simulink model "WindFarmDFIG"  (R2024a)
settings: Solver=FixedStepDiscrete  StartTime=0.0  StopTime=0.2  RelTol=1e-3
PreLoadFcn:
  | Ts=5e-6;
InitFcn:
  | xInitial = WindFarmDFIGInit;
  | Ts=5e-6;
undefined symbols (not defined in the file): D1, D11, Delta, DiscIntNeverNeededParam, find_system, level
libraries: powerlib_extras x38, spsThreePhaseVIMeasurementLib x6, simulink_extras x6, spsThreePhaseTransformerTwoWindingsLib x3, spsSeriesRLCBranchLib x2, spsUniversalBridgeLib x2, spsGroundLib x2, spsThreePhaseProgrammableVoltageSourceLib x1, spsThreePhaseMutualInductanceZ1Z0Lib x1, spsThreePhasePISectionLineLib x1, spsAsynchronousMachinepuUnitsLib x1, spsThreePhaseSeriesRLCBranchLib x1
(part 2 of 3)

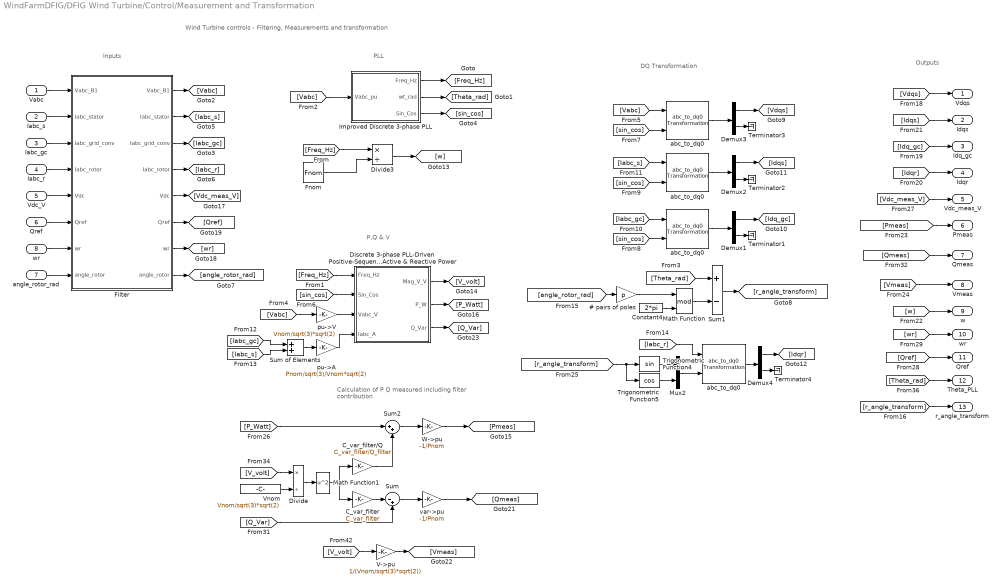
== system WindFarmDFIG/DFIG Wind Turbine/Control/Measurement and Transformation ==
  note: DQ Transformation
  note: P,Q & V
  note: PLL
  note: Inputs
  note: Outputs
  note: Calculation of P Q measured
      | including filter contribution
  note: Wind Turbine controls - Filtering, Measurements and transformation
  Vabc : Inport
  Iabc_s : Inport  Port=2
  Iabc_gc : Inport  Port=3
  Iabc_r : Inport  Port=4
  Vdc_V : Inport  Port=5
  Qref : Inport  Port=6
  angle_rotor_rad : Inport  Port=7
  wr : Inport  Port=8
  "   abc_to_dq0    " : powerlib_extras/Measurements/abc_to_dq0 Transformation
  " Improved Discrete 3-phase PLL" : Subsystem  mask(Discrete 3-phase PLL){Fmin=0.75*Fnom, Par_Init=[0 Fnom], ParK=[5 3.2 1 50], Ts=Ts}
      mask prompts: Fmin "Minimum frequency (Hz):"; Par_Init "Initial inputs:[ Phase(degrees)   Frequency(Hz) ]"; ParK "Regulator gains [ Kp1 Kp2  Ki1  Ki2 ]"; Ts "Sample time:"
      mask help:
      | This Phase Locked Loop (PLL) system can be used  to synchronize on a set of variable frequency, three-phase sinusoidal signals.
      |
      | Input 1: Vector containing the normalized
      |              three-phase signals [Va Vb Vc]
      | Output 1:  Measured frequency (Hz) = w/(2pi)
      | Output 2:  Ramp w.t   varying between  0 and 2*pi,
      | synchronized on zero crossings of the fundamental (positive-sequence) of phase A.
      | Output 3: Vector [sin(wt) cos(wt)]
      mask init:
      | Kp1=ParK(1);
      | Kp2=ParK(2);
      | Ki1=ParK(3);
      | Ki2=ParK(4);
      | Phase_Init=Par_Init(1);
      | Finit=Par_Init(2);
      | power_initmask();
      settings: OpenFcn=power_openblockproxy();
  # pairs of poles : Gain  Gain=p  SaturateOnIntegerOverflow=on  OutDataTypeStr=Inherit: Same as input  ParamDataTypeStr=Inherit: Same as input
  C_var_filter : Gain  Gain=C_var_filter  SaturateOnIntegerOverflow=on  OutDataTypeStr=Inherit: Same as input  ParamDataTypeStr=Inherit: Same as input
  C_var_filter/Q : Gain  Gain=C_var_filter/Q_filter  SaturateOnIntegerOverflow=on  OutDataTypeStr=Inherit: Same as input  ParamDataTypeStr=Inherit: Same as input
  Constant4 : Constant  Value=2*pi
  Demux{1..4} (4 alike) : Demux  Outputs=[2 1]
      settings: DisplayOption=none
  Discrete 3-phase PLL-Driven Positive-Sequence Active & Reactive Power : Subsystem  mask(Discrete 3-phase PLL-Driven Positive-Sequence Active & Reactive Power){Finit=Fnom, Fmin=Fnom*45/60, Par_Vinit=[Vnom/sqrt(3)*sqrt(2) 30], Par_Iinit=[Pnom/sqrt(3)/Vnom*sqrt(2) -10], Ts=Ts}
      mask prompts: Finit "Initial frequency (Hz):"; Fmin "Minimum frequency (Hz):"; Par_Vinit "Voltage initial input: [ Mag  Phase(Degrees) ]"; Par_Iinit "Current initial input: [ Mag  Phase(Degrees) ]"; Ts "Sample time:"
      mask help:
      | This discrete block measures the 3-phase active power P and reactive power Q  associated with a periodic set of 3-phase voltages and currents which may contain harmonics. P and Q are calculated by evaluating the fundamental values (positive-sequence) of the input voltages and currents with a running window over one cycle of the specified frequency (port Freq).
      |  Input port "Sin_Cos" (a two-dimension signal) provides the reference frame required for the computation.
      |
      | input 1: must give the frequency of the fundamental (Hz)
      | Input 2: must contain a  [sin(wt)  cos(wt)] two dimension signal , where w is the rotation speed (rad/s) of the reference frame used for the computation..
      | input 3: Vectorized 3-phase  instantaneous voltage (Vabc)
      | input 4: Vectorized 3-phase instantaneous current (Iabc)
      |
      | Output 1: Vector [Mag_V Mag_I] of the fundamental values (Magnitude) of the voltage & current (peak values of the positive-sequence)
      | Output 2: 3-phase PQ measurement vector [P(W) Q (var)] evaluated at the specified frequency. Current flowing into an RL circuit will produce  positive active and reactive powers.
      |
      | For the first cycle of simulation, the outputs are held constant using the values specified by the parameters "Initial input".
      | he value of the parameter "Minimum frequency" is used to determine the buffer size of the "Variable Transport Delay" block found inside this subsystem.
      mask init:
      | power_initmask();
      settings: OpenFcn=power_openblockproxy();
  Divide : Product  Inputs=*/
  Divide3 : Product  Inputs=*/
  Filter : Subsystem  mask{Freq=Freq_filter, Zeta1=Zeta_filter, Ts=Ts}
      mask prompts: Freq "Cut-off frequency (Hz):"; Zeta1 "Damping factor Zeta:"; Ts "Sample time"
  Fnom : Constant  Value=Fnom
  Math Function : Math  Operator=mod  SignedPower=on
  Math Function1 : Math  Operator=square  SignedPower=on
  Mux2 : Mux  Inputs=2
  Sum : Sum  Inputs=|-+
  Sum of Elements : Sum
  Sum1 : Sum  Inputs=+-  InputSameDT=on  SaturateOnIntegerOverflow=on  OutDataTypeStr=Inherit: Same as first input
  Sum2 : Sum  Inputs=|++
  Terminator{1..4} (4 alike) : Terminator
  Trigonometric Function4 : Trigonometry
  Trigonometric Function5 : Trigonometry  Operator=cos
  V->pu : Gain  Gain=1/(Vnom/sqrt(3)*sqrt(2))  SaturateOnIntegerOverflow=on  OutDataTypeStr=Inherit: Same as input  ParamDataTypeStr=Inherit: Same as input
  Vnom : Constant  Value=Vnom/sqrt(3)*sqrt(2)
  W->pu : Gain  Gain=-1/Pnom  SaturateOnIntegerOverflow=on  OutDataTypeStr=Inherit: Same as input  ParamDataTypeStr=Inherit: Same as input
  abc_to_dq0 : powerlib_extras/Measurements/abc_to_dq0 Transformation
  "abc_to_dq0 " : powerlib_extras/Measurements/abc_to_dq0 Transformation
  "abc_to_dq0  " : powerlib_extras/Measurements/abc_to_dq0 Transformation
  pu->A : Gain  Gain=Pnom/sqrt(3)/Vnom*sqrt(2)  SaturateOnIntegerOverflow=on  OutDataTypeStr=Inherit: Same as input  ParamDataTypeStr=Inherit: Same as input
  pu->V : Gain  Gain=Vnom/sqrt(3)*sqrt(2)  SaturateOnIntegerOverflow=on  OutDataTypeStr=Inherit: Same as input  ParamDataTypeStr=Inherit: Same as input
  "var->pu " : Gain  Gain=-1/Pnom  SaturateOnIntegerOverflow=on  OutDataTypeStr=Inherit: Same as input  ParamDataTypeStr=Inherit: Same as input
  Vdqs : Outport  VectorParamsAs1DForOutWhenUnconnected=off
  Idqs : Outport  Port=2  VectorParamsAs1DForOutWhenUnconnected=off
  Idq_gc : Outport  Port=3  VectorParamsAs1DForOutWhenUnconnected=off
  Idqr : Outport  Port=4  VectorParamsAs1DForOutWhenUnconnected=off
  Vdc_meas_V : Outport  Port=5  VectorParamsAs1DForOutWhenUnconnected=off
  Pmeas : Outport  Port=6  VectorParamsAs1DForOutWhenUnconnected=off
  Qmeas : Outport  Port=7  VectorParamsAs1DForOutWhenUnconnected=off
  Vmeas : Outport  Port=8  VectorParamsAs1DForOutWhenUnconnected=off
  w : Outport  Port=9  VectorParamsAs1DForOutWhenUnconnected=off
  "wr " : Outport  Port=10  VectorParamsAs1DForOutWhenUnconnected=off
  "Qref " : Outport  Port=11  VectorParamsAs1DForOutWhenUnconnected=off
  Theta_PLL : Outport  Port=12  VectorParamsAs1DForOutWhenUnconnected=off
  r_angle_transform : Outport  Port=13  VectorParamsAs1DForOutWhenUnconnected=off
  wires:
  " Improved Discrete 3-phase PLL"/3(Sin_Cos) -> [sin_cos]
  " Improved Discrete 3-phase PLL"/2(wt_rad) -> [Theta_rad]
  " Improved Discrete 3-phase PLL"/1(Freq_Hz) -> [Freq_Hz]
  [Vabc] -> " Improved Discrete 3-phase PLL"/1(Vabc_pu)
  [r_angle_transform] -> r_angle_transform/1
  [V_volt] -> V->pu/1
  V->pu/1 -> [Vmeas]
  [Theta_rad] -> Theta_PLL/1
  [Qmeas] -> Qmeas/1
  Discrete 3-phase PLL-Driven Positive-Sequence Active & Reactive Power/2(P_W) -> [P_Watt]
  Discrete 3-phase PLL-Driven Positive-Sequence Active & Reactive Power/1(Mag_V_V) -> [V_volt]
  Demux1/2 -> Terminator1/1
  Demux3/1 -> [Vdqs]
  Demux3/2 -> Terminator3/1
  "abc_to_dq0  "/1 -> Demux1/1
  abc_to_dq0/1 -> Demux3/1
  Math Function/1 -> Sum1/2
  # pairs of poles/1 -> Math Function/1
  Constant4/1 -> Math Function/2
  Demux4/1 -> [Idqr]
  Demux4/2 -> Terminator4/1
  "   abc_to_dq0    "/1 -> Demux4/1
  Demux2/2 -> Terminator2/1
  Trigonometric Function5/1 -> Mux2/2
  Trigonometric Function4/1 -> Mux2/1
  "abc_to_dq0 "/1 -> Demux2/1
  Fnom/1 -> Divide3/2
  Divide3/1 -> [w]
  Sum of Elements/1 -> pu->A/1
  pu->V/1 -> Discrete 3-phase PLL-Driven Positive-Sequence Active & Reactive Power/3(Vabc_V)
  [Freq_Hz] -> Divide3/1
  [Freq_Hz] -> Discrete 3-phase PLL-Driven Positive-Sequence Active & Reactive Power/1(Freq_Hz)
  [Vabc] -> pu->V/1
  [Vabc] -> abc_to_dq0/1
  [sin_cos] -> Discrete 3-phase PLL-Driven Positive-Sequence Active & Reactive Power/2(Sin_Cos)
  [sin_cos] -> abc_to_dq0/2
  [sin_cos] -> "abc_to_dq0  "/2
  [sin_cos] -> "abc_to_dq0 "/2
  [angle_rotor_rad] -> # pairs of poles/1
  [Iabc_gc] -> "abc_to_dq0  "/1
  [Iabc_s] -> "abc_to_dq0 "/1
  [Iabc_s] -> Sum of Elements/2
  [Iabc_r] -> "   abc_to_dq0    "/1
  Demux1/1 -> [Idq_gc]
  Demux2/1 -> [Idqs]
  [Vdqs] -> Vdqs/1
  [Idq_gc] -> Idq_gc/1
  [Idqr] -> Idqr/1
  [Idqs] -> Idqs/1
  [w] -> w/1
  [Pmeas] -> Pmeas/1
  [Vmeas] -> Vmeas/1
  pu->A/1 -> Discrete 3-phase PLL-Driven Positive-Sequence Active & Reactive Power/4(Iabc_A)
  Sum1/1 -> [r_angle_transform]
  Mux2/1 -> "   abc_to_dq0    "/2
  [r_angle_transform] -> Trigonometric Function4/1, Trigonometric Function5/1
  Vabc/1 -> Filter/1(Vabc_B1)
  Iabc_s/1 -> Filter/2(Iabc_stator)
  Iabc_gc/1 -> Filter/3(Iabc_grid_conv)
  Iabc_r/1 -> Filter/4(Iabc_rotor)
  Vdc_V/1 -> Filter/5(Vdc)
  Qref/1 -> Filter/6(Qref)
  wr/1 -> Filter/7(wr)
  [Vdc_meas_V] -> Vdc_meas_V/1
  [Qref] -> "Qref "/1
  [wr] -> "wr "/1
  "var->pu "/1 -> [Qmeas]
  [Q_Var] -> Sum/2
  W->pu/1 -> [Pmeas]
  [P_Watt] -> Sum2/1
  [V_volt] -> Divide/1
  Vnom/1 -> Divide/2
  Divide/1 -> Math Function1/1
  C_var_filter/1 -> Sum/1
  Sum/1 -> "var->pu "/1
  C_var_filter/Q/1 -> Sum2/2
  Sum2/1 -> W->pu/1
  Math Function1/1 -> C_var_filter/Q/1, C_var_filter/1
  Filter/1("Vabc_B1 ") -> [Vabc]
  Filter/2("Iabc_stator ") -> [Iabc_s]
  Filter/3("Iabc_grid_conv ") -> [Iabc_gc]
  Filter/4("Iabc_rotor ") -> [Iabc_r]
  Filter/5("Vdc ") -> [Vdc_meas_V]
  Filter/6("Qref ") -> [Qref]
  Filter/7("wr ") -> [wr]
  Filter/8("angle_rotor ") -> [angle_rotor_rad]
  angle_rotor_rad/1 -> Filter/8(angle_rotor)
  [Iabc_gc] -> Sum of Elements/1
  Discrete 3-phase PLL-Driven Positive-Sequence Active & Reactive Power/3(Q_Var) -> [Q_Var]
  [Theta_rad] -> Sum1/1

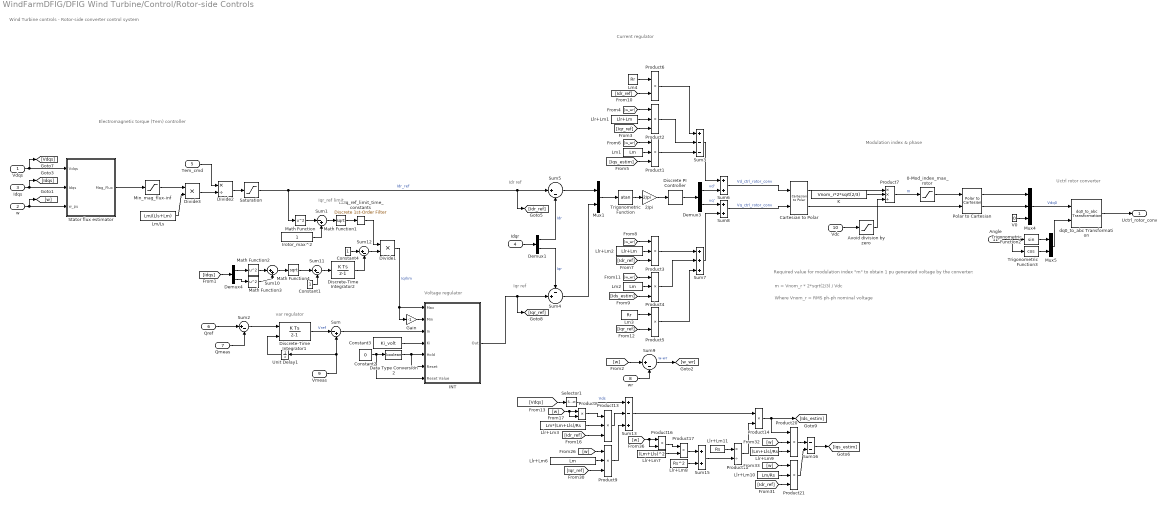
== system WindFarmDFIG/DFIG Wind Turbine/Control/Rotor-side Controls ==
  note: Uctrl rotor converter
  note: Modulation index & phase
  note: Required value for modulation index "m" to obtain 1 pu generated voltage by the converter:
  note: m = Vnom_r * 2*sqrt(2/3) / Vdc
  note: Where Vnom_r = RMS ph-ph nominal voltage
  note: Current regulator
  note: Electromagnetic torque (Tem) controller
  note: Wind Turbine controls - Rotor-side converter control system
  note: Iqr ref
  note: Idr ref
  note: Iqr_ref limit
  note: Voltage regulator
  note: var regulator
  Vdqs : Inport
  w : Inport  Port=2
  Idqs : Inport  Port=3
  Idqr : Inport  Port=4
  Tem_cmd : Inport  Port=5
  Qref : Inport  Port=6
  Qmeas : Inport  Port=7
  wr : Inport  Port=8
  Vmeas : Inport  Port=9
  Vdc : Inport  Port=10
  Angle : Inport  Port=11
  0-Mod_index_max_rotor : Saturate  UpperLimit=Mod_index_max_rotor  LowerLimit=0
  2/pi : Gain  Gain=2/pi
  Avoid division by zero : Saturate  UpperLimit=inf  LowerLimit=1e-6
  Cartesian to Polar : simulink_extras/Transformations/Cartesian to Polar
  Constant1 : Constant
  Constant2 : Constant  Value=0
  Constant3 : Constant  Value=Ki_volt
  Constant4 : Constant
  Data Type Conversion2 : DataTypeConversion  OutDataTypeStr=boolean  SaturateOnIntegerOverflow=off  RndMeth=Floor
  Demux1 : Demux  Outputs=2
      settings: DisplayOption=none
  Demux3 : Demux  Outputs=2
      settings: DisplayOption=none
  Demux4 : Demux  Outputs=2
      settings: DisplayOption=none
  Discrete PI Controller : powerlib_extras/Discrete  Control Blocks/Discrete PI Controller  Kp=Kp_rotor_side_cur_reg  Ki=Ki_rotor_side_cur_reg  Par_Limits=[1 -1]*Lim_rotor_side_cur_reg  Init=0  Ts=Ts
  Discrete-Time Integrator1 : DiscreteIntegrator  gainval=Ki_var  InitialConditionSource=external  InitialCondition=1  SampleTime=Ts  LimitOutput=on  UpperSaturationLimit=Max_var_reg  LowerSaturationLimit=Min_var_reg  ICPrevOutput=DiscIntNeverNeededParam  ICPrevScaledInput=DiscIntNeverNeededParam
  Discrete-Time Integrator2 : DiscreteIntegrator  gainval=10  SampleTime=Ts  LimitOutput=on  UpperSaturationLimit=1  LowerSaturationLimit=0  ICPrevOutput=DiscIntNeverNeededParam  ICPrevScaledInput=DiscIntNeverNeededParam
  Divide1 : Product  Inputs=**
  Divide2 : Product  Inputs=*/
  Divide3 : Product  Inputs=**
  Gain : Gain  Gain=-1  SaturateOnIntegerOverflow=on  OutDataTypeStr=Inherit: Same as input  ParamDataTypeStr=Inherit: Same as input
  INT : Subsystem  mask(Integrator  With  External  Dynamic  Limits (Discrete)){}
      mask Display: disp('Discrete-Time\n(Trapezoidal)\nIntegrator\n ')
  Irotor_max^2 : Constant
  K : Constant  Value=Vnom_r*2*sqrt(2/3)
  Llr+Lm1 : Constant  Value=Llr+Lm
  Llr+Lm10 : Constant  Value=Lm/Rs
  Llr+Lm11 : Constant  Value=Rs
  Llr+Lm2 : Constant  Value=Llr+Lm
  Llr+Lm3 : Constant  Value=Lm*(Lm+Lls)/Rs
  Llr+Lm6 : Constant  Value=Lm
  Llr+Lm7 : Constant  Value=(Lm+Lls)^2
  Llr+Lm8 : Constant  Value=Rs^2
  Llr+Lm9 : Constant  Value=(Lm+Lls)/Rs
  Lm/Ls : Constant  Value=Lm/(Lls+Lm)
  Lm1 : Constant  Value=Lm
  Lm2 : Constant  Value=Lm
  Lm3 : Constant  Value=Rr
  Lm4 : Constant  Value=Rr  VectorParams1D=off
  Math Function : Math  Operator=square  SignedPower=on
  Math Function1 : Math  Operator=sqrt  SignedPower=on
  Math Function2 : Math  Operator=square  SignedPower=on
  Math Function3 : Math  Operator=square  SignedPower=on
  Math Function4 : Math  Operator=sqrt  SignedPower=on
  Min_mag_flux-inf : Saturate  UpperLimit=inf  LowerLimit=Min_mag_flux
  Mux1 : Mux  Inputs=2
  Mux4 : Mux  Inputs=3
  Mux5 : Mux  Inputs=2
  Polar to Cartesian : simulink_extras/Transformations/Polar to Cartesian
  Product{1..4,9,13,20..21} (8 alike) : Product  Inputs=3  SaturateOnIntegerOverflow=on  OutDataTypeStr=Inherit: Same as first input
  Product{5..6,8,14,16..17} (6 alike) : Product  SaturateOnIntegerOverflow=on  OutDataTypeStr=Inherit: Same as first input
  Product18 : Product  Inputs=*/  SaturateOnIntegerOverflow=on  OutDataTypeStr=Inherit: Same as first input
  Product7 : Product  Inputs=**/  InputSameDT=on  SaturateOnIntegerOverflow=on  OutDataTypeStr=Inherit: Same as first input
  Saturation : Saturate  UpperLimit=Max_Idr_ref  LowerLimit=0
  Selector1 : Selector  InputPortWidth=2  IndexOptions=Index vector (dialog)  Indices=1  OutputSizes=[(-2)]
  Stator flux estimator : Subsystem
  Sum : Sum  Inputs=|-+  InputSameDT=on  SaturateOnIntegerOverflow=on  OutDataTypeStr=Inherit: Same as first input
  Sum1 : Sum  Inputs=|-+  InputSameDT=on  SaturateOnIntegerOverflow=on  OutDataTypeStr=Inherit: Same as first input
  Sum10 : Sum  Inputs=|++  InputSameDT=on  SaturateOnIntegerOverflow=on  OutDataTypeStr=Inherit: Same as first input
  Sum{2,5,9,11..12} (5 alike) : Sum  Inputs=|+-  InputSameDT=on  SaturateOnIntegerOverflow=on  OutDataTypeStr=Inherit: Same as first input
  Sum13 : Sum  Inputs=+-+  InputSameDT=on  SaturateOnIntegerOverflow=on  OutDataTypeStr=Inherit: Same as first input
  Sum15 : Sum  InputSameDT=on  SaturateOnIntegerOverflow=on  OutDataTypeStr=Inherit: Same as first input
  Sum16 : Sum  Inputs=--  InputSameDT=on  SaturateOnIntegerOverflow=on  OutDataTypeStr=Inherit: Same as first input
  Sum3 : Sum  Inputs=+--  InputSameDT=on  SaturateOnIntegerOverflow=on  OutDataTypeStr=Inherit: Same as first input
  Sum4 : Sum  Inputs=-+|  InputSameDT=on  SaturateOnIntegerOverflow=on  OutDataTypeStr=Inherit: Same as first input
  Sum6 : Sum  InputSameDT=on  SaturateOnIntegerOverflow=on  OutDataTypeStr=Inherit: Same as first input
  Sum7 : Sum  Inputs=+++  InputSameDT=on  SaturateOnIntegerOverflow=on  OutDataTypeStr=Inherit: Same as first input
  Sum8 : Sum  InputSameDT=on  SaturateOnIntegerOverflow=on  OutDataTypeStr=Inherit: Same as first input
  Trigonometric Function : Trigonometry  Operator=atan
  Trigonometric Function2 : Trigonometry
  Trigonometric Function3 : Trigonometry  Operator=cos
  Unit Delay1 : UnitDelay  InitialCondition=1  SampleTime=Ts  HasFrameUpgradeWarning=on
  V0 : Constant  Value=0
  dq0_to_abc Transformation : powerlib_extras/Measurements/dq0_to_abc Transformation
  t=Iq_ref_limit_time_constants : powerlib_extras/Discrete  Control Blocks/Discrete 1st-Order Filter  FilterType=Lowpass  Tc=Iq_ref_limit_time_constant  Ts=Ts  Initialize=on  Vac_Init=[0 0 0]  Vdc_Init=Imax_grid_conv  PlotResponse=off  param1=[1 500 0.1]
  Uctrl_rotor_conv : Outport  VectorParamsAs1DForOutWhenUnconnected=off
  wires:
  Demux4/2 -> Math Function3/1
  Demux4/1 -> Math Function2/1
  Sum16/1 -> [Iqs_estim]
  [Vdqs] -> Selector1/1
  Selector1/1 -> Sum13/1  "Vds"
  [w] -> Product8/1, Product8/2
  Product8/1 -> Product13/1
  Llr+Lm3/1 -> Product13/2
  [Idr_ref] -> Product13/3
  Llr+Lm6/1 -> Product9/2
  [Iqr_ref] -> Product9/3
  [w] -> Product9/1
  Product13/1 -> Sum13/2
  Product9/1 -> Sum13/3
  Sum13/1 -> Product14/1
  [w] -> Product16/2, Product16/1
  Product16/1 -> Product17/1
  Llr+Lm7/1 -> Product17/2
  Product17/1 -> Sum15/1
  Llr+Lm10/1 -> Product21/2
  [w] -> Product21/1
  [Idr_ref] -> Product21/3
  Product20/1 -> Sum16/1
  Product21/1 -> Sum16/2
  Llr+Lm8/1 -> Sum15/2
  Sum15/1 -> Product18/2
  Llr+Lm11/1 -> Product18/1
  Product18/1 -> Product14/2
  Product14/1 -> [Ids_estim], Product20/1
  Llr+Lm9/1 -> Product20/3
  [w] -> Product20/2
  Sum12/1 -> Divide1/2
  Divide1/1 -> Gain/1, INT/1(Max)  "Iqrlim"
  Sum11/1 -> Discrete-Time Integrator2/1
  Constant4/1 -> Sum12/1
  Discrete-Time Integrator2/1 -> Sum12/2
  t=Iq_ref_limit_time_constants/1 -> Divide1/1
  Constant1/1 -> Sum11/2
  Math Function4/1 -> Sum11/1
  Sum10/1 -> Math Function4/1
  Math Function3/1 -> Sum10/2
  Math Function2/1 -> Sum10/1
  0-Mod_index_max_rotor/1 -> Polar to Cartesian/1
  Polar to Cartesian/2 -> Mux4/2
  Polar to Cartesian/1 -> Mux4/1
  Cartesian to Polar/2 -> Polar to Cartesian/2
  Product7/1 -> 0-Mod_index_max_rotor/1  "m"
  INT/1(Out) -> [Iqr_ref], Sum4/2
  Sum8/1 -> Cartesian to Polar/2  "Vq_ctrl_rotor_conv"
  Sum6/1 -> Cartesian to Polar/1  "Vd_ctrl_rotor_conv"
  Vdc/1 -> Avoid division by zero/1
  Avoid division by zero/1 -> Product7/3
  Mux4/1 -> dq0_to_abc Transformation/1  "Vdq0"
  V0/1 -> Mux4/3
  dq0_to_abc Transformation/1 -> Uctrl_rotor_conv/1
  Angle/1 -> Trigonometric Function3/1, Trigonometric Function2/1
  Trigonometric Function3/1 -> Mux5/2
  Trigonometric Function2/1 -> Mux5/1
  Mux5/1 -> dq0_to_abc Transformation/2
  K/1 -> Product7/2
  Cartesian to Polar/1 -> Product7/1
  Idqr/1 -> Demux1/1
  wr/1 -> Sum9/2
  Sum9/1 -> [w_wr]  "w-wr"
  [w] -> Sum9/1
  [Idqs] -> Demux4/1
  Sum5/1 -> Mux1/1
  Sum4/1 -> Mux1/2
  Demux1/1 -> Sum5/2  "Idr"
  Demux1/2 -> Sum4/1  "Iqr"
  Mux1/1 -> Trigonometric Function/1
  Trigonometric Function/1 -> 2/pi/1
  2/pi/1 -> Discrete PI Controller/1
  [w_wr] -> Product2/1
  Llr+Lm1/1 -> Product2/2
  [Iqs_estim] -> Product1/3
  [w_wr] -> Product1/1
  Lm1/1 -> Product1/2
  Lm4/1 -> Product6/1
  Product1/1 -> Sum3/3
  [Idr_ref] -> Product6/2
  [Iqr_ref] -> Product2/3
  Product6/1 -> Sum3/1
  Product2/1 -> Sum3/2
  [w_wr] -> Product3/1
  Llr+Lm2/1 -> Product3/2
  [Ids_estim] -> Product4/3
  [w_wr] -> Product4/1
  Lm2/1 -> Product4/2
  Product4/1 -> Sum7/2
  Lm3/1 -> Product5/1
  [Iqr_ref] -> Product5/2
  [Idr_ref] -> Product3/3
  Product3/1 -> Sum7/1
  Product5/1 -> Sum7/3
  Discrete PI Controller/1 -> Demux3/1
  Demux3/1 -> Sum6/2  "vd'"
  Demux3/2 -> Sum8/1  "vq'"
  Sum3/1 -> Sum6/1
  Sum7/1 -> Sum8/2
  Vmeas/1 -> Unit Delay1/1, Sum/2
  Qmeas/1 -> Sum2/2
  Qref/1 -> Sum2/1
  Sum2/1 -> Discrete-Time Integrator1/1
  Unit Delay1/1 -> Discrete-Time Integrator1/2
  Math Function/1 -> Sum1/1
  Irotor_max^2/1 -> Sum1/2
  Sum1/1 -> Math Function1/1
  Math Function1/1 -> t=Iq_ref_limit_time_constants/1
  Discrete-Time Integrator1/1 -> Sum/1  "Vref"
  Constant3/1 -> INT/4(Ki)
  Gain/1 -> INT/2(Min)
  Data Type Conversion2/1 -> INT/6(Reset), INT/5(Hold)
  Constant2/1 -> INT/7(Reset Value), Data Type Conversion2/1
  Sum/1 -> INT/3(In)
  Saturation/1 -> [Idr_ref], Sum5/1, Math Function/1  "Idr_ref"
  Tem_cmd/1 -> Divide2/1
  Idqs/1 -> Stator flux estimator/2(Idqs), [Idqs]
  Vdqs/1 -> [Vdqs], Stator flux estimator/1(Vdqs)
  Divide3/1 -> Divide2/2
  Divide2/1 -> Saturation/1
  Lm/Ls/1 -> Divide3/2
  Min_mag_flux-inf/1 -> Divide3/1
  Stator flux estimator/1(Mag_Flux) -> Min_mag_flux-inf/1
  w/1 -> Stator flux estimator/3(w_pu), [w]

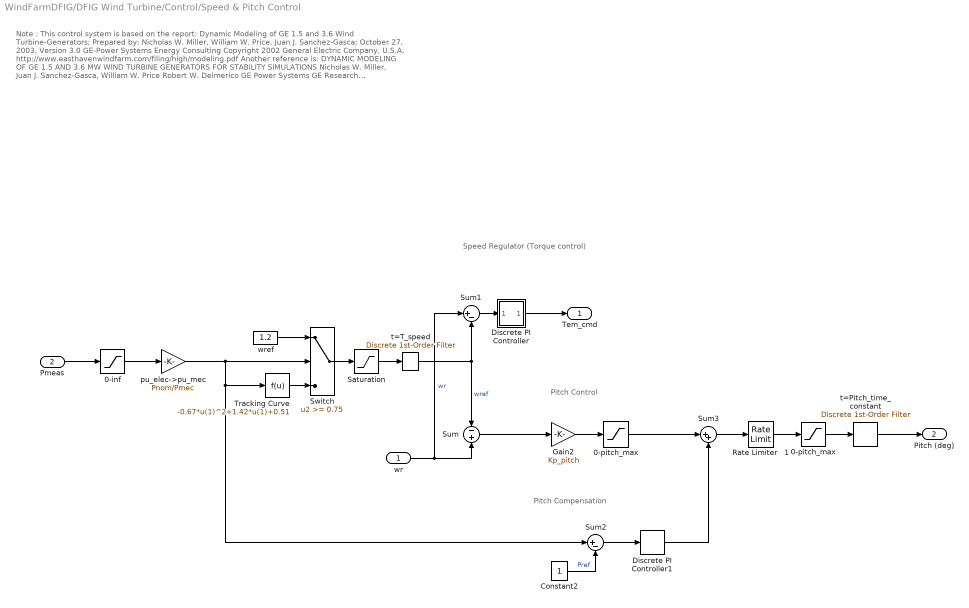
== system WindFarmDFIG/DFIG Wind Turbine/Control/Speed & Pitch Control ==
  note: Note :
      | This control system is based on the report:
      | Dynamic Modeling of GE 1.5 and 3.6 Wind Turbine-Generators;
      | Prepared by: Nicholas W. Miller, William W. Price, Juan J. Sanchez-Gasca;
      | October 27, 2003, Version 3.0
      | GE-Power Systems Energy Consulting
      | Copyright 2002 General Electric Company, U.S.A.
      |
      | http://www.easthavenwindfarm.com/filing/high/modeling.pdf
      |
      | Another reference is:
      |
      | DYNAMIC MODELING OF GE 1.5 AND 3.6 MW WIND TURBINE GENERATORS
      | FOR STABILITY SIMULATIONS
      | Nicholas W. Miller, Juan J. Sanchez-Gasca, William W. Price Robert W. Delmerico
      | GE Power Systems GE Research
      | Schenectady, NY Niskayuna, NY
      |
      | 0-7803-7989-6/03/$17.00 02003 IEEE
  note: Speed Regulator
      | (Torque control)
  note: Pitch Compensation
  note: Pitch Control
  wr : Inport
  Pmeas : Inport  Port=2
  0-inf : Saturate  UpperLimit=inf  LowerLimit=0
  0-pitch_max : Saturate  UpperLimit=pitch_max  LowerLimit=0
  "0-pitch_max " : Saturate  UpperLimit=pitch_max  LowerLimit=0
  Constant2 : Constant
  Discrete PI Controller : Subsystem  DialogController=POWERSYS.PowerSysDialog  mask(Discrete PI Controller){Kp=Kp_speed, Ki=Ki_speed, Par_Limits=[Max_speed_reg 0], Init=0.7, Ts=Ts}
      mask prompts: Kp "Proportional gain (Kp):"; Ki "Integral gain (Ki):"; Par_Limits "Output limits: [ Upper   Lower ]"; Init "Output initial value:"; Ts "Sample time:"
      mask help: This block implements a discrete PI controller.
      mask init:
      | UpperLimit=Par_Limits(1);
      | LowerLimit=Par_Limits(2);
      | power_initmask();
      mask Help: This block is part of a subset of blocks in the Extras library that does not have documentation associated with it, other than the block mask description.
      mask Display: disp('PI');
  Discrete PI Controller1 : powerlib_extras/Discrete  Control Blocks/Discrete PI Controller  Kp=Kp_compensation  Ki=Ki_compensation  Par_Limits=[pitch_max 0]  Init=0  Ts=Ts
  Gain2 : Gain  Gain=Kp_pitch  SaturateOnIntegerOverflow=on  OutDataTypeStr=Inherit: Same as input  ParamDataTypeStr=Inherit: Same as input
  Rate Limiter   1 : RateLimiter  RisingSlewLimit=pitch_rate  FallingSlewLimit=-pitch_rate
  Saturation : Saturate  UpperLimit=Speed_max  LowerLimit=Speed_min
  Sum : Sum  Inputs=-+  SaturateOnIntegerOverflow=on
  Sum1 : Sum  Inputs=|+-
  Sum2 : Sum  Inputs=|+-  SaturateOnIntegerOverflow=on
  Sum3 : Sum  Inputs=|++
  Switch : Switch  Threshold=0.75  SaturateOnIntegerOverflow=off  InputSameDT=off
  Tracking Curve : Fcn  Expr=-0.67*u(1)^2+1.42*u(1)+0.51
  pu_elec->pu_mec : Gain  Gain=Pnom/Pmec
  t=Pitch_time_constant : powerlib_extras/Discrete  Control Blocks/Discrete 1st-Order Filter  FilterType=Lowpass  Tc=Pitch_time_constant  Ts=Ts  Initialize=on  Vac_Init=[0.8 -25 60]*0  Vdc_Init=0  PlotResponse=off  param1=[1 500 0.1]
  t=T_speed : powerlib_extras/Discrete  Control Blocks/Discrete 1st-Order Filter  FilterType=Lowpass  Tc=T_speed  Ts=Ts  Initialize=on  Vac_Init=[0 0 0]  Vdc_Init=1-init(1)  PlotResponse=off  param1=[1 500 0.1]
  wref : Constant  Value=1.2
  Tem_cmd : Outport  VectorParamsAs1DForOutWhenUnconnected=off
  Pitch (deg) : Outport  Port=2  VectorParamsAs1DForOutWhenUnconnected=off
  wires:
  Saturation/1 -> t=T_speed/1
  wref/1 -> Switch/1
  Tracking Curve/1 -> Switch/3
  Discrete PI Controller/1(Out) -> Tem_cmd/1
  t=T_speed/1 -> Sum/1, Sum1/2  "wref"
  Sum2/1 -> Discrete PI Controller1/1
  t=Pitch_time_constant/1 -> Pitch (deg)/1
  Sum/1 -> Gain2/1
  "0-pitch_max "/1 -> t=Pitch_time_constant/1
  0-pitch_max/1 -> Sum3/1
  Pmeas/1 -> 0-inf/1
  Discrete PI Controller1/1 -> Sum3/2
  Gain2/1 -> 0-pitch_max/1
  Rate Limiter   1/1 -> "0-pitch_max "/1
  Sum3/1 -> Rate Limiter   1/1
  Constant2/1 -> Sum2/2  "Pref"
  Sum1/1 -> Discrete PI Controller/1(Error)
  Switch/1 -> Saturation/1
  pu_elec->pu_mec/1 -> Switch/2, Tracking Curve/1, Sum2/1
  0-inf/1 -> pu_elec->pu_mec/1
  wr/1 -> Sum/2, Sum1/1  "wr"

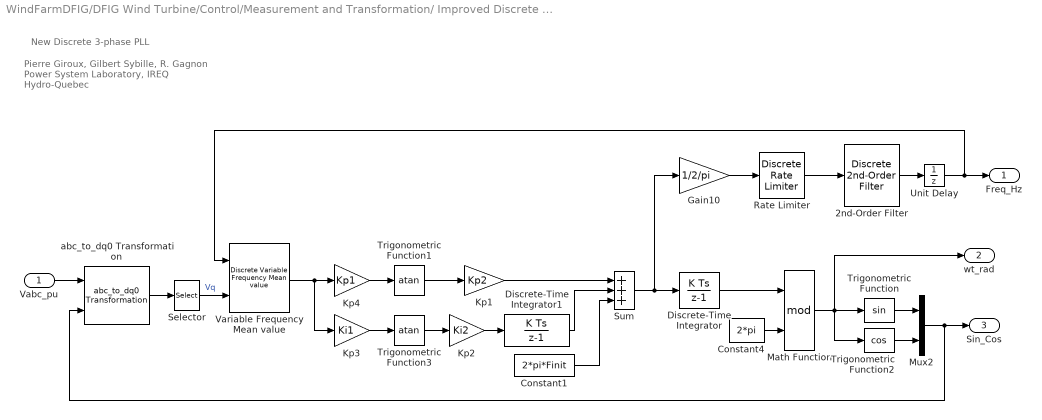
== system WindFarmDFIG/DFIG Wind Turbine/Control/Measurement and Transformation/ Improved Discrete 3-phase PLL ==
  note: Pierre Giroux, Gilbert Sybille, R. Gagnon
      | Power System Laboratory, IREQ
      | Hydro-Quebec
  note: New Discrete 3-phase PLL
  Vabc_pu : Inport  PortDimensions=3
  2nd-Order Filter : powerlib_extras/Discrete  Control Blocks/Discrete  2nd-Order Filter  FilterType=Lowpass  Fo=25  Zeta=0.707  Ts=Ts  Initialize=on  Vac_Init=[0 0 Finit]  Vdc_Init=Finit  PlotResponse=off  param1=[1 500 0.1]
  Constant1 : Constant  Value=2*pi*Finit
  Constant4 : Constant  Value=2*pi
  Discrete-Time Integrator : DiscreteIntegrator  SampleTime=Ts  ICPrevOutput=DiscIntNeverNeededParam  ICPrevScaledInput=DiscIntNeverNeededParam
  Discrete-Time Integrator1 : DiscreteIntegrator  gainval=1  SampleTime=Ts  LimitOutput=on  UpperSaturationLimit=2*pi*5  LowerSaturationLimit=-2*pi*5  ICPrevOutput=DiscIntNeverNeededParam  ICPrevScaledInput=DiscIntNeverNeededParam
  Gain10 : Gain  Gain=1/2/pi  SaturateOnIntegerOverflow=on  OutDataTypeStr=Inherit: Same as input  ParamDataTypeStr=Inherit: Same as input
  Kp1 : Gain  Gain=Kp2  SaturateOnIntegerOverflow=on  OutDataTypeStr=Inherit: Same as input  ParamDataTypeStr=Inherit: Same as input
  Kp2 : Gain  Gain=Ki2  SaturateOnIntegerOverflow=on  OutDataTypeStr=Inherit: Same as input  ParamDataTypeStr=Inherit: Same as input
  Kp3 : Gain  Gain=Ki1  SaturateOnIntegerOverflow=on  OutDataTypeStr=Inherit: Same as input  ParamDataTypeStr=Inherit: Same as input
  Kp4 : Gain  Gain=Kp1  SaturateOnIntegerOverflow=on  OutDataTypeStr=Inherit: Same as input  ParamDataTypeStr=Inherit: Same as input
  Math Function : Math  Operator=mod  SignedPower=on
  Mux2 : Mux  Inputs=2
  Rate Limiter : powerlib_extras/Discrete  Control Blocks/Discrete Rate Limiter  R=12  F=-12  Vinit=Finit  Ts=Ts
  Selector : Selector  InputPortWidth=3  IndexOptions=Index vector (dialog)  Indices=2  OutputSizes=1
  Sum : Sum  Inputs=+++
  Trigonometric Function : Trigonometry
  Trigonometric Function1 : Trigonometry  Operator=atan
  Trigonometric Function2 : Trigonometry  Operator=cos
  Trigonometric Function3 : Trigonometry  Operator=atan
  Unit Delay : UnitDelay  InitialCondition=Finit  SampleTime=Ts  HasFrameUpgradeWarning=on
  Variable Frequency Mean value : powerlib_extras/Discrete Measurements/Discrete Variable Frequency Mean value  Finit=Finit  Fmin=Fmin  Vinit=0  Ts=Ts
  abc_to_dq0 Transformation : powerlib_extras/Measurements/abc_to_dq0 Transformation
  Freq_Hz : Outport  VectorParamsAs1DForOutWhenUnconnected=off
  wt_rad : Outport  Port=2  VectorParamsAs1DForOutWhenUnconnected=off
  Sin_Cos : Outport  Port=3  VectorParamsAs1DForOutWhenUnconnected=off
  wires:
  Discrete-Time Integrator1/1 -> Sum/2
  Kp1/1 -> Sum/1
  Discrete-Time Integrator/1 -> Math Function/1
  Unit Delay/1 -> Variable Frequency Mean value/1, Freq_Hz/1
  Sum/1 -> Gain10/1, Discrete-Time Integrator/1
  Kp2/1 -> Discrete-Time Integrator1/1
  Trigonometric Function3/1 -> Kp2/1
  Kp3/1 -> Trigonometric Function3/1
  Variable Frequency Mean value/1 -> Kp3/1, Kp4/1
  Constant1/1 -> Sum/3
  Trigonometric Function1/1 -> Kp1/1
  Kp4/1 -> Trigonometric Function1/1
  Selector/1 -> Variable Frequency Mean value/2  "Vq"
  2nd-Order Filter/1 -> Unit Delay/1
  Rate Limiter/1 -> 2nd-Order Filter/1
  Gain10/1 -> Rate Limiter/1
  Mux2/1 -> abc_to_dq0 Transformation/2, Sin_Cos/1
  Trigonometric Function2/1 -> Mux2/2
  Trigonometric Function/1 -> Mux2/1
  Math Function/1 -> wt_rad/1, Trigonometric Function2/1, Trigonometric Function/1
  Constant4/1 -> Math Function/2
  abc_to_dq0 Transformation/1 -> Selector/1
  Vabc_pu/1 -> abc_to_dq0 Transformation/1

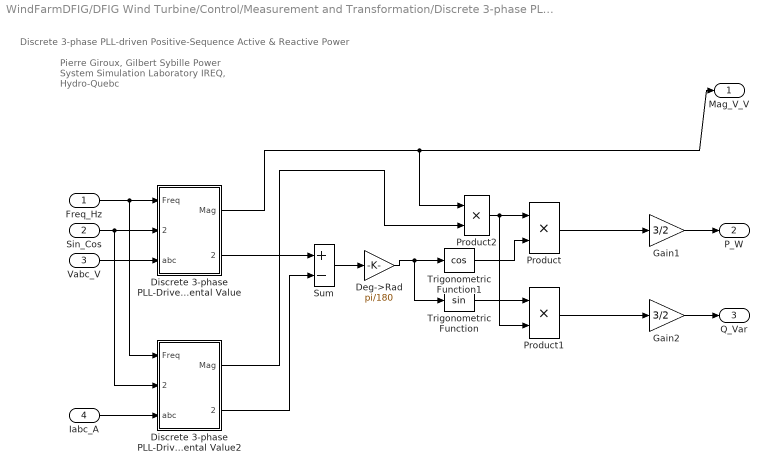
== system WindFarmDFIG/DFIG Wind Turbine/Control/Measurement and Transformation/Discrete 3-phase PLL-Driven Positive-Sequence Active & Reactive Power ==
  note: Discrete 3-phase PLL-driven Positive-Sequence Active & Reactive Power
  note: Pierre Giroux, Gilbert Sybille
      | Power System Simulation Laboratory
      | IREQ, Hydro-Quebc
  Freq_Hz : Inport  PortDimensions=1
  Sin_Cos : Inport  Port=2  PortDimensions=2
  Vabc_V : Inport  Port=3  PortDimensions=3
  Iabc_A : Inport  Port=4  PortDimensions=3
  Deg->Rad : Gain  Gain=pi/180  SaturateOnIntegerOverflow=on  OutDataTypeStr=Inherit: Same as input  ParamDataTypeStr=Inherit: Same as input
  Discrete 3-phase PLL-Driven Positive-Sequence Fundamental Value : Subsystem  mask(Discrete 3-phase PLL-Driven Positive-Sequence Fundamental Value){Finit=Finit, Fmin=Fmin, Par_Init=Par_Vinit, Ts=Ts}
      mask prompts: Finit "Initial frequency (Hz):"; Fmin "Minimum frequency (Hz):"; Par_Init "Initial input (positive component): [ Mag  Phase-relative-to-PLL(degrees) ]"; Ts "Sample time:"
      mask help:
      | For a supplied fundamental frequency (port Freq), this discrete block computes  the positive-sequence component (Magnitude and Phase)  of a set of three balanced or unbalanced signals (port abc) which may contain harmonics.
      |  Input port "Sin_Cos" (a two-dimension signal) provides the reference frame required for the computation..
      |  First and second outputs return respectively the magnitude and phase (in degrees relative to the PLL phase)) of the fundamental.
      | For the first cycle of simulation, the outputs are held constant to the values specified by the parameter "Initial input".
      | constant to the values specified by the parameter "Initial input". The value of the parameter "Minimum frequency" is used to determine the buffer size of the "Variable Transport Delay" block found inside this subsystem.
      mask init:
      | Real_Init=Par_Init(1)*cos(pi/180*Par_Init(2));
      | Imag_Init=Par_Init(1)*sin(pi/180*Par_Init(2));
      | power_initmask();
      settings: OpenFcn=power_openblockproxy();
  Discrete 3-phase PLL-Driven Positive-Sequence Fundamental Value2 : Subsystem  mask(Discrete 3-phase PLL-Driven Positive-Sequence Fundamental Value){Finit=Finit, Fmin=Fmin, Par_Init=Par_Iinit, Ts=Ts}
      mask prompts: Finit "Initial frequency (Hz):"; Fmin "Minimum frequency (Hz):"; Par_Init "Initial input (positive component): [ Mag  Phase-relative-to-PLL(degrees) ]"; Ts "Sample time:"
      mask help:
      | For a supplied fundamental frequency (port Freq), this discrete block computes  the positive-sequence component (Magnitude and Phase)  of a set of three balanced or unbalanced signals (port abc) which may contain harmonics.
      |  Input port "Sin_Cos" (a two-dimension signal) provides the reference frame required for the computation..
      |  First and second outputs return respectively the magnitude and phase (in degrees relative to the PLL phase)) of the fundamental.
      | For the first cycle of simulation, the outputs are held constant to the values specified by the parameter "Initial input".
      | constant to the values specified by the parameter "Initial input". The value of the parameter "Minimum frequency" is used to determine the buffer size of the "Variable Transport Delay" block found inside this subsystem.
      mask init:
      | Real_Init=Par_Init(1)*cos(pi/180*Par_Init(2));
      | Imag_Init=Par_Init(1)*sin(pi/180*Par_Init(2));
      | power_initmask();
      settings: OpenFcn=power_openblockproxy();
  Gain1 : Gain  Gain=3/2  SaturateOnIntegerOverflow=on  OutDataTypeStr=Inherit: Same as input  ParamDataTypeStr=Inherit: Same as input
  Gain2 : Gain  Gain=3/2  SaturateOnIntegerOverflow=on  OutDataTypeStr=Inherit: Same as input  ParamDataTypeStr=Inherit: Same as input
  Product : Product  InputSameDT=on  SaturateOnIntegerOverflow=on  OutDataTypeStr=Inherit: Same as first input
  Product1 : Product  InputSameDT=on  SaturateOnIntegerOverflow=on  OutDataTypeStr=Inherit: Same as first input
  Product2 : Product  InputSameDT=on  SaturateOnIntegerOverflow=on  OutDataTypeStr=Inherit: Same as first input
  Sum : Sum  Inputs=+-  InputSameDT=on  SaturateOnIntegerOverflow=on  OutDataTypeStr=Inherit: Same as first input
  Trigonometric Function : Trigonometry
  Trigonometric Function1 : Trigonometry  Operator=cos
  Mag_V_V : Outport  VectorParamsAs1DForOutWhenUnconnected=off
  P_W : Outport  Port=2  VectorParamsAs1DForOutWhenUnconnected=off
  Q_Var : Outport  Port=3  VectorParamsAs1DForOutWhenUnconnected=off
  wires:
  Vabc_V/1 -> Discrete 3-phase PLL-Driven Positive-Sequence Fundamental Value/3(abc)
  Freq_Hz/1 -> Discrete 3-phase PLL-Driven Positive-Sequence Fundamental Value/1(Freq), Discrete 3-phase PLL-Driven Positive-Sequence Fundamental Value2/1(Freq)
  Sin_Cos/1 -> Discrete 3-phase PLL-Driven Positive-Sequence Fundamental Value/2(Sin_Cos), Discrete 3-phase PLL-Driven Positive-Sequence Fundamental Value2/2(Sin_Cos)
  Discrete 3-phase PLL-Driven Positive-Sequence Fundamental Value/2(Phase) -> Sum/1
  Discrete 3-phase PLL-Driven Positive-Sequence Fundamental Value/1(Mag) -> Product2/1, Mag_V_V/1
  Discrete 3-phase PLL-Driven Positive-Sequence Fundamental Value2/2(Phase) -> Sum/2
  Sum/1 -> Deg->Rad/1
  Deg->Rad/1 -> Trigonometric Function1/1, Trigonometric Function/1
  Trigonometric Function1/1 -> Product/2
  Trigonometric Function/1 -> Product1/1
  Product/1 -> Gain1/1
  Gain1/1 -> P_W/1
  Product2/1 -> Product/1, Product1/2
  Discrete 3-phase PLL-Driven Positive-Sequence Fundamental Value2/1(Mag) -> Product2/2
  Iabc_A/1 -> Discrete 3-phase PLL-Driven Positive-Sequence Fundamental Value2/3(abc)
  Product1/1 -> Gain2/1
  Gain2/1 -> Q_Var/1

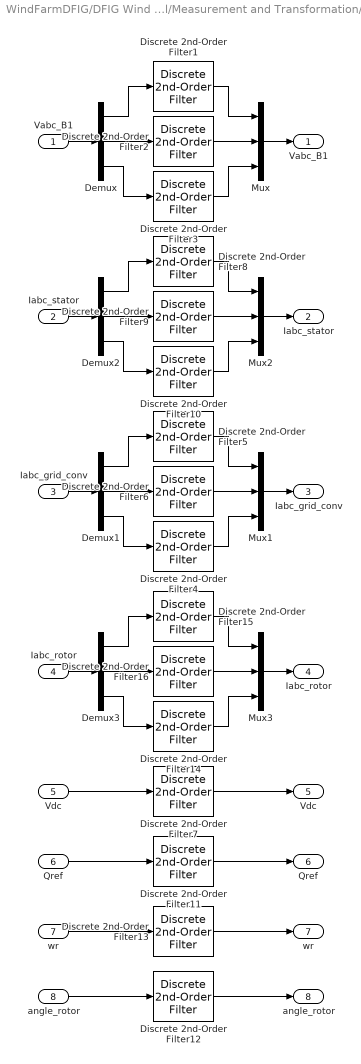
== system WindFarmDFIG/DFIG Wind Turbine/Control/Measurement and Transformation/Filter ==
  Vabc_B1 : Inport
  Iabc_stator : Inport  Port=2
  Iabc_grid_conv : Inport  Port=3
  Iabc_rotor : Inport  Port=4
  Vdc : Inport  Port=5
  Qref : Inport  Port=6
  wr : Inport  Port=7
  angle_rotor : Inport  Port=8
  Demux{,1..3} (4 alike) : Demux  Outputs=3
      settings: DisplayOption=none
  Discrete 2nd-Order Filter{1..6,8..16} (15 alike) : powerlib_extras/Discrete  Control Blocks/Discrete  2nd-Order Filter  FilterType=Lowpass  Fo=Freq  Zeta=Zeta1  Ts=Ts  Initialize=off  Vac_Init=[0.8 -25 60]  Vdc_Init=-0.4  PlotResponse=off  param1=[1 500 1]
  Discrete 2nd-Order Filter7 : powerlib_extras/Discrete  Control Blocks/Discrete  2nd-Order Filter  FilterType=Lowpass  Fo=Freq  Zeta=Zeta1  Ts=Ts  Initialize=on  Vac_Init=[0.8 -25 60]*0  Vdc_Init=Vdc_nom  PlotResponse=off  param1=[1 500 1]
  Mux{,1..3} (4 alike) : Mux  Inputs=3
  "Vabc_B1 " : Outport  VectorParamsAs1DForOutWhenUnconnected=off
  "Iabc_stator " : Outport  Port=2  VectorParamsAs1DForOutWhenUnconnected=off
  "Iabc_grid_conv " : Outport  Port=3  VectorParamsAs1DForOutWhenUnconnected=off
  "Iabc_rotor " : Outport  Port=4  VectorParamsAs1DForOutWhenUnconnected=off
  "Vdc " : Outport  Port=5  VectorParamsAs1DForOutWhenUnconnected=off
  "Qref " : Outport  Port=6  VectorParamsAs1DForOutWhenUnconnected=off
  "wr " : Outport  Port=7  VectorParamsAs1DForOutWhenUnconnected=off
  "angle_rotor " : Outport  Port=8  VectorParamsAs1DForOutWhenUnconnected=off
  wires:
  Demux/1 -> Discrete 2nd-Order Filter1/1
  Demux/2 -> Discrete 2nd-Order Filter2/1
  Demux/3 -> Discrete 2nd-Order Filter3/1
  Discrete 2nd-Order Filter1/1 -> Mux/1
  Discrete 2nd-Order Filter2/1 -> Mux/2
  Discrete 2nd-Order Filter3/1 -> Mux/3
  Vabc_B1/1 -> Demux/1
  Mux/1 -> "Vabc_B1 "/1
  Demux1/1 -> Discrete 2nd-Order Filter5/1
  Demux1/2 -> Discrete 2nd-Order Filter6/1
  Demux1/3 -> Discrete 2nd-Order Filter4/1
  Discrete 2nd-Order Filter5/1 -> Mux1/1
  Discrete 2nd-Order Filter6/1 -> Mux1/2
  Discrete 2nd-Order Filter4/1 -> Mux1/3
  Iabc_grid_conv/1 -> Demux1/1
  Mux1/1 -> "Iabc_grid_conv "/1
  Vdc/1 -> Discrete 2nd-Order Filter7/1
  Discrete 2nd-Order Filter7/1 -> "Vdc "/1
  Demux2/1 -> Discrete 2nd-Order Filter8/1
  Demux2/2 -> Discrete 2nd-Order Filter9/1
  Demux2/3 -> Discrete 2nd-Order Filter10/1
  Discrete 2nd-Order Filter8/1 -> Mux2/1
  Discrete 2nd-Order Filter9/1 -> Mux2/2
  Discrete 2nd-Order Filter10/1 -> Mux2/3
  Iabc_stator/1 -> Demux2/1
  Mux2/1 -> "Iabc_stator "/1
  wr/1 -> Discrete 2nd-Order Filter13/1
  Discrete 2nd-Order Filter13/1 -> "wr "/1
  Demux3/1 -> Discrete 2nd-Order Filter15/1
  Demux3/2 -> Discrete 2nd-Order Filter16/1
  Demux3/3 -> Discrete 2nd-Order Filter14/1
  Discrete 2nd-Order Filter15/1 -> Mux3/1
  Discrete 2nd-Order Filter16/1 -> Mux3/2
  Discrete 2nd-Order Filter14/1 -> Mux3/3
  Iabc_rotor/1 -> Demux3/1
  Mux3/1 -> "Iabc_rotor "/1
  Qref/1 -> Discrete 2nd-Order Filter11/1
  Discrete 2nd-Order Filter11/1 -> "Qref "/1
  angle_rotor/1 -> Discrete 2nd-Order Filter12/1
  Discrete 2nd-Order Filter12/1 -> "angle_rotor "/1

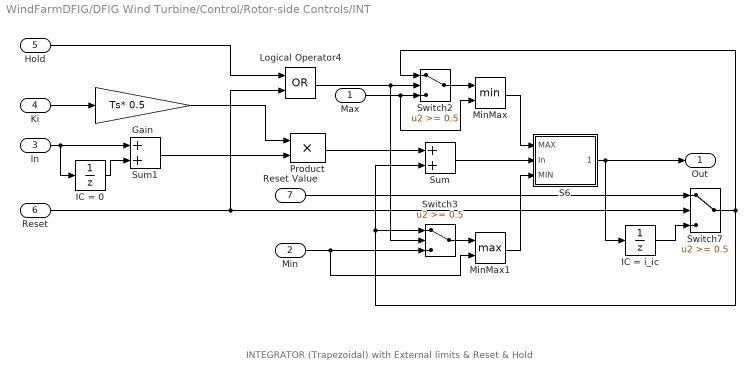
== system WindFarmDFIG/DFIG Wind Turbine/Control/Rotor-side Controls/INT ==
  note: INTEGRATOR (Trapezoidal) with External limits & Reset & Hold
  Max : Inport
  Min : Inport  Port=2
  In : Inport  Port=3
  Ki : Inport  Port=4
  Hold : Inport  Port=5
  Reset : Inport  Port=6
  Reset Value : Inport  Port=7
  Gain : Gain  Gain=Ts* 0.5  SaturateOnIntegerOverflow=on  OutDataTypeStr=Inherit: Same as input  ParamDataTypeStr=Inherit: Same as input
  IC = 0 : UnitDelay  SampleTime=Ts  HasFrameUpgradeWarning=on
  IC = i_ic : UnitDelay  SampleTime=Ts  HasFrameUpgradeWarning=on
  Logical Operator4 : Logic  Operator=OR
  MinMax : MinMax  Inputs=2  InputSameDT=on  SaturateOnIntegerOverflow=on
  MinMax1 : MinMax  Function=max  Inputs=2  InputSameDT=on  SaturateOnIntegerOverflow=on
  Product : Product  SaturateOnIntegerOverflow=on  OutDataTypeStr=Inherit: Same as first input
  S6 : Subsystem  mask(Limiter with External Limits){}
      mask Display: disp('      Limiter\n')
  Sum : Sum  InputSameDT=on  SaturateOnIntegerOverflow=on  OutDataTypeStr=Inherit: Same as first input
  Sum1 : Sum  InputSameDT=on  SaturateOnIntegerOverflow=on  OutDataTypeStr=Inherit: Same as first input
  Switch2 : Switch  Threshold=0.5
  Switch3 : Switch  Threshold=0.5
  Switch7 : Switch  Threshold=0.5
  Out : Outport  InitialOutput=0  VectorParamsAs1DForOutWhenUnconnected=off
  wires:
  S6/1("  ") -> IC = i_ic/1, Out/1
  Gain/1 -> Product/1
  Sum1/1 -> Product/2
  Ki/1 -> Gain/1
  IC = 0/1 -> Sum1/2
  In/1 -> IC = 0/1, Sum1/1
  Product/1 -> Sum/1
  Sum/1 -> S6/2(In)
  Hold/1 -> Logical Operator4/1
  Reset/1 -> Switch7/2, Logical Operator4/2
  Logical Operator4/1 -> Switch2/2, Switch3/2
  Switch2/1 -> MinMax/1
  Max/1 -> Switch2/3, MinMax/2
  Reset Value/1 -> Switch7/1
  MinMax/1 -> S6/1(MAX)
  MinMax1/1 -> S6/3(MIN)
  Switch3/1 -> MinMax1/1
  Min/1 -> Switch3/3, MinMax1/2
  IC = i_ic/1 -> Switch7/3
  Switch7/1 -> Switch2/1, Sum/2, Switch3/1

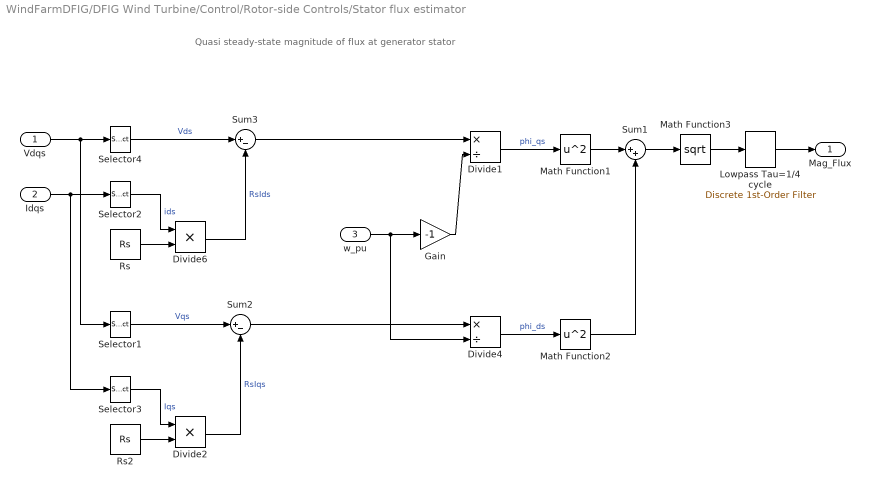
== system WindFarmDFIG/DFIG Wind Turbine/Control/Rotor-side Controls/Stator flux estimator ==
  note: Quasi steady-state magnitude of flux at generator stator
  Vdqs : Inport
  Idqs : Inport  Port=2
  w_pu : Inport  Port=3
  Divide1 : Product  Inputs=*/
  Divide2 : Product  Inputs=**
  Divide4 : Product  Inputs=*/
  Divide6 : Product  Inputs=**
  Gain : Gain  Gain=-1
  Lowpass Tau=1/4 cycle : powerlib_extras/Discrete  Control Blocks/Discrete 1st-Order Filter  FilterType=Lowpass  Tc=0.25*(1/Fnom)  Ts=Ts  Initialize=on  Vac_Init=[0.8 -25 60]*0  Vdc_Init=1  PlotResponse=off  param1=[1 500 0.1]
  Math Function1 : Math  Operator=square  SignedPower=on
  Math Function2 : Math  Operator=square  SignedPower=on
  Math Function3 : Math  Operator=sqrt  SignedPower=on
  Rs : Constant  Value=Rs
  Rs2 : Constant  Value=Rs
  Selector1 : Selector  InputPortWidth=2  IndexOptions=Index vector (dialog)  Indices=2  OutputSizes=1
  Selector2 : Selector  InputPortWidth=2  IndexOptions=Index vector (dialog)  Indices=1  OutputSizes=1
  Selector3 : Selector  InputPortWidth=2  IndexOptions=Index vector (dialog)  Indices=2  OutputSizes=1
  Selector4 : Selector  InputPortWidth=2  IndexOptions=Index vector (dialog)  Indices=1  OutputSizes=1
  Sum1 : Sum  Inputs=|++
  Sum2 : Sum  Inputs=|+-
  Sum3 : Sum  Inputs=|+-
  Mag_Flux : Outport  VectorParamsAs1DForOutWhenUnconnected=off
  wires:
  Math Function2/1 -> Sum1/2
  Divide4/1 -> Math Function2/1  "phi_ds"
  Sum2/1 -> Divide4/1
  Divide2/1 -> Sum2/2  "RsIqs"
  Rs2/1 -> Divide2/2
  Selector3/1 -> Divide2/1  "Iqs"
  Selector1/1 -> Sum2/1  "Vqs"
  Math Function3/1 -> Lowpass Tau=1/4 cycle/1
  Sum1/1 -> Math Function3/1
  Math Function1/1 -> Sum1/1
  Divide1/1 -> Math Function1/1  "phi_qs"
  Gain/1 -> Divide1/2
  Sum3/1 -> Divide1/1
  w_pu/1 -> Divide4/2, Gain/1
  Selector4/1 -> Sum3/1  "Vds"
  Vdqs/1 -> Selector1/1, Selector4/1
  Rs/1 -> Divide6/2
  Selector2/1 -> Divide6/1  "ids"
  Divide6/1 -> Sum3/2  "RsIds"
  Idqs/1 -> Selector3/1, Selector2/1
  Lowpass Tau=1/4 cycle/1 -> Mag_Flux/1

== system WindFarmDFIG/DFIG Wind Turbine/Control/Speed & Pitch Control/Discrete PI Controller ==
  note: Discrete PID Controller
  note: Pierre Giroux, Gilbert Sybille
      | Power System Simulation Laboratory
      | IREQ, Hydro-Quebc
  Error : Inport
  Discrete-Time Integrator : DiscreteIntegrator  InitialCondition=Init  SampleTime=Ts  LimitOutput=on  UpperSaturationLimit=UpperLimit  LowerSaturationLimit=LowerLimit  ICPrevOutput=DiscIntNeverNeededParam  ICPrevScaledInput=DiscIntNeverNeededParam
  Product1 : Product  RndMeth=Zero
  Product2 : Product  RndMeth=Zero
  Saturation2 : Saturate  UpperLimit=UpperLimit  LowerLimit=LowerLimit
  Step_Ki_speed : Step  Time=999  Before=Ki  After=Ki  SampleTime=Ts
  Step_Kp_speed : Step  Time=999  Before=Kp  After=Kp  SampleTime=Ts
  Sum6 : Sum  InputSameDT=on  SaturateOnIntegerOverflow=on  OutDataTypeStr=Inherit: Same as first input
  Out : Outport  InitialOutput=0  VectorParamsAs1DForOutWhenUnconnected=off
  wires:
  Saturation2/1 -> Out/1
  Discrete-Time Integrator/1 -> Sum6/2
  Product1/1 -> Sum6/1
  Product2/1 -> Discrete-Time Integrator/1
  Sum6/1 -> Saturation2/1
  Error/1 -> Product1/2, Product2/1
  Step_Kp_speed/1 -> Product1/1
  Step_Ki_speed/1 -> Product2/2

== system WindFarmDFIG/DFIG Wind Turbine/Control/Measurement and Transformation/Discrete 3-phase PLL-Driven Positive-Sequence Active & Reactive Power/Discrete 3-phase PLL-Driven Positive-Sequence Fundamental Value ==
  note: Discrete 3-phase PLL-Driven Positive-Sequence Fundamental Value
  note: Pierre Giroux, Gilbert Sybille
      | Power System Simulation Laboratory
      | IREQ, Hydro-Quebc
  Freq : Inport
  Sin_Cos : Inport  Port=2  PortDimensions=2
  abc : Inport  Port=3  PortDimensions=3
  Cartesian to Polar : simulink_extras/Transformations/Cartesian to Polar
  Demux : Demux  Outputs=3
      settings: DisplayOption=none
  Discrete Variable Frequency Mean value1 : Subsystem  mask(Discrete Variable-Frequency Mean Value){Finit=Finit, Fmin=Fmin, Vinit=Imag_Init, Ts=Ts}
      mask prompts: Finit "Initial frequency (Hz):"; Fmin "Minimum frequency (Hz):"; Vinit "Initial input (DC component):"; Ts "Sample time:"
      mask help:
      | This discrete block computes the mean value of the input signal (port In) over a running window of one cycle of a specified frequency (port Freq).
      |
      | For the first cycle of simulation (specified by the parameter "Initial frequency"), the output is held to the value of the  "Initial input" parameter.
      |
      | The value of the parameter "Minimum frequency" is used to determine the buffer size of the "Variable Transport Delay" block found inside this subsystem.
      mask init:
      | MaxDelay=1/Fmin+Ts;
      | power_initmask();
      settings: OpenFcn=power_openblockproxy();
  Discrete Variable Frequency Mean value2 : Subsystem  mask(Discrete Variable-Frequency Mean Value){Finit=Finit, Fmin=Fmin, Vinit=Real_Init, Ts=Ts}
      mask prompts: Finit "Initial frequency (Hz):"; Fmin "Minimum frequency (Hz):"; Vinit "Initial input (DC component):"; Ts "Sample time:"
      mask help:
      | This discrete block computes the mean value of the input signal (port In) over a running window of one cycle of a specified frequency (port Freq).
      |
      | For the first cycle of simulation (specified by the parameter "Initial frequency"), the output is held to the value of the  "Initial input" parameter.
      |
      | The value of the parameter "Minimum frequency" is used to determine the buffer size of the "Variable Transport Delay" block found inside this subsystem.
      mask init:
      | MaxDelay=1/Fmin+Ts;
      | power_initmask();
      settings: OpenFcn=power_openblockproxy();
  Rad->Deg. : Gain  Gain=180/pi  SaturateOnIntegerOverflow=on  OutDataTypeStr=Inherit: Same as input  ParamDataTypeStr=Inherit: Same as input
  Terminator : Terminator
  abc_to_dq0 Transformation : powerlib_extras/Measurements/abc_to_dq0 Transformation
  Mag : Outport  VectorParamsAs1DForOutWhenUnconnected=off
  Phase : Outport  Port=2  VectorParamsAs1DForOutWhenUnconnected=off
  wires:
  Cartesian to Polar/2 -> Rad->Deg./1
  Cartesian to Polar/1 -> Mag/1
  Demux/3 -> Terminator/1
  abc_to_dq0 Transformation/1 -> Demux/1
  abc/1 -> abc_to_dq0 Transformation/1
  Demux/1 -> Discrete Variable Frequency Mean value2/2(In)
  Demux/2 -> Discrete Variable Frequency Mean value1/2(In)
  Discrete Variable Frequency Mean value1/1(Mean) -> Cartesian to Polar/2  "Real"
  Rad->Deg./1 -> Phase/1
  Discrete Variable Frequency Mean value2/1(Mean) -> Cartesian to Polar/1  "Real"
  Freq/1 -> Discrete Variable Frequency Mean value1/1(Freq), Discrete Variable Frequency Mean value2/1(Freq)
  Sin_Cos/1 -> abc_to_dq0 Transformation/2

== system WindFarmDFIG/DFIG Wind Turbine/Control/Measurement and Transformation/Discrete 3-phase PLL-Driven Positive-Sequence Active & Reactive Power/Discrete 3-phase PLL-Driven Positive-Sequence Fundamental Value2 ==
  note: Pierre Giroux, Gilbert Sybille
      | Power System Simulation Laboratory
      | IREQ, Hydro-Quebc
  note: Discrete 3-phase PLL-Driven Positive-Sequence Fundamental Value
  Freq : Inport
  Sin_Cos : Inport  Port=2  PortDimensions=2
  abc : Inport  Port=3  PortDimensions=3
  Cartesian to Polar : simulink_extras/Transformations/Cartesian to Polar
  Demux : Demux  Outputs=3
      settings: DisplayOption=none
  Discrete Variable Frequency Mean value1 : Subsystem  mask(Discrete Variable-Frequency Mean Value){Finit=Finit, Fmin=Fmin, Vinit=Imag_Init, Ts=Ts}
      mask prompts: Finit "Initial frequency (Hz):"; Fmin "Minimum frequency (Hz):"; Vinit "Initial input (DC component):"; Ts "Sample time:"
      mask help:
      | This discrete block computes the mean value of the input signal (port In) over a running window of one cycle of a specified frequency (port Freq).
      |
      | For the first cycle of simulation (specified by the parameter "Initial frequency"), the output is held to the value of the  "Initial input" parameter.
      |
      | The value of the parameter "Minimum frequency" is used to determine the buffer size of the "Variable Transport Delay" block found inside this subsystem.
      mask init:
      | MaxDelay=1/Fmin+Ts;
      | power_initmask();
      settings: OpenFcn=power_openblockproxy();
  Discrete Variable Frequency Mean value2 : Subsystem  mask(Discrete Variable-Frequency Mean Value){Finit=Finit, Fmin=Fmin, Vinit=Real_Init, Ts=Ts}
      mask prompts: Finit "Initial frequency (Hz):"; Fmin "Minimum frequency (Hz):"; Vinit "Initial input (DC component):"; Ts "Sample time:"
      mask help:
      | This discrete block computes the mean value of the input signal (port In) over a running window of one cycle of a specified frequency (port Freq).
      |
      | For the first cycle of simulation (specified by the parameter "Initial frequency"), the output is held to the value of the  "Initial input" parameter.
      |
      | The value of the parameter "Minimum frequency" is used to determine the buffer size of the "Variable Transport Delay" block found inside this subsystem.
      mask init:
      | MaxDelay=1/Fmin+Ts;
      | power_initmask();
      settings: OpenFcn=power_openblockproxy();
  Rad->Deg. : Gain  Gain=180/pi  SaturateOnIntegerOverflow=on  OutDataTypeStr=Inherit: Same as input  ParamDataTypeStr=Inherit: Same as input
  Terminator : Terminator
  abc_to_dq0 Transformation : powerlib_extras/Measurements/abc_to_dq0 Transformation
  Mag : Outport  VectorParamsAs1DForOutWhenUnconnected=off
  Phase : Outport  Port=2  VectorParamsAs1DForOutWhenUnconnected=off
  wires:
  Sin_Cos/1 -> abc_to_dq0 Transformation/2
  Freq/1 -> Discrete Variable Frequency Mean value2/1(Freq), Discrete Variable Frequency Mean value1/1(Freq)
  Discrete Variable Frequency Mean value2/1(Mean) -> Cartesian to Polar/1  "Real"
  Rad->Deg./1 -> Phase/1
  Discrete Variable Frequency Mean value1/1(Mean) -> Cartesian to Polar/2  "Real"
  Demux/2 -> Discrete Variable Frequency Mean value1/2(In)
  Demux/1 -> Discrete Variable Frequency Mean value2/2(In)
  abc/1 -> abc_to_dq0 Transformation/1
  abc_to_dq0 Transformation/1 -> Demux/1
  Demux/3 -> Terminator/1
  Cartesian to Polar/1 -> Mag/1
  Cartesian to Polar/2 -> Rad->Deg./1

== system WindFarmDFIG/DFIG Wind Turbine/Control/Rotor-side Controls/INT/S6 ==
  note: Limiter
      | with external
      | limits
  MAX : Inport
  In : Inport  Port=2
  MIN : Inport  Port=3
  MinMax : MinMax  Function=max  Inputs=2  InputSameDT=on  SaturateOnIntegerOverflow=on
  MinMax1 : MinMax  Inputs=2  InputSameDT=on  SaturateOnIntegerOverflow=on
  "  " : Outport  InitialOutput=0  VectorParamsAs1DForOutWhenUnconnected=off
  wires:
  In/1 -> MinMax1/2
  MinMax/1 -> "  "/1
  MIN/1 -> MinMax/1
  MAX/1 -> MinMax1/1
  MinMax1/1 -> MinMax/2
